simulink model "gnc_uav_toolbox_DCIntegration"  (R2025b)
settings: Solver=FixedStepAuto  StartTime=0  StopTime=cfg.stopTime  MaxStep=0.01  RelTol=1e-5
values from neighbouring files (symbols this model uses):
  C = [cfg.kPos;cfg.vNom;cfg.vMax;cfg.landSpeed;cfg.aMax ... (first row only)    [gn_init.m]    (also in gnc_init_dcintegration.m = [cfg.kPos;cfg.vNom;cfg.vMax;cfg.landSpeed;cfg.aMax;       cf; smooth_path.m = q(:, c) - Lt(c)*x + r*y)
  entryPoint = S(1,:).'    [gn_buildSearch.m]    (also in gn_build_mission.m = mission.p_end(:, 2))
  homeAir = [cfg.home(1); cfg.home(2); -cfg.altitude]    [gn_buildSearch.m]    (also in gn_build_mission.m = mission.p_end(:, 1))
  lastPoint = S(end,:).'    [gn_buildSearch.m]    (also in gn_build_mission.m = mission.p_end(:, 3))
  searchW = [wp(:, 2:n); -cfg.altitude*ones(1, n-1)]'    [gn_build_mission.m]
undefined symbols (not defined in the file or in its folder): cfg, DiscIntNeverNeededParam
libraries: uavalgslib x1, uavutilslib x1
settings Model: Creator=andrei  LastModifiedBy=andrei
settings OptimizationCC: OptimizeBlockIOStorage=off  ZeroExternalMemoryAtStartup=off  ZeroInternalMemoryAtStartup=off  OptimizeDataStoreBuffers=off  BusAssignmentInplaceUpdate=off
settings DebuggingCC: SFUnexpectedBacktrackingDiag=warning  SFNoUnconditionalDefaultTransitionDiag=warning
settings RTWCC: GenerateReport=on  BuildConfiguration=Debug  LaunchReport=on  TargetLang=C++
settings CodeAppCC: ForceParamTrailComments=on  MATLABSourceComments=on  EnableCustomComments=on
settings GRTTargetCC: MultiInstanceErrorCode=Warning  TargetLangStandard=C++11 (ISO)  CombineSignalStateStructs=on  CodeInterfacePackaging=C++ class  SubcomponentCodeInterfacePackaging=C++ class  SupportVariableSizeSignals=on

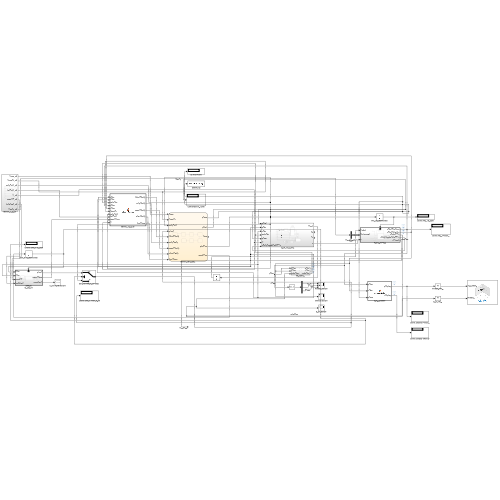
[thumbnail: Simulink's stored preview of the top-level diagram]
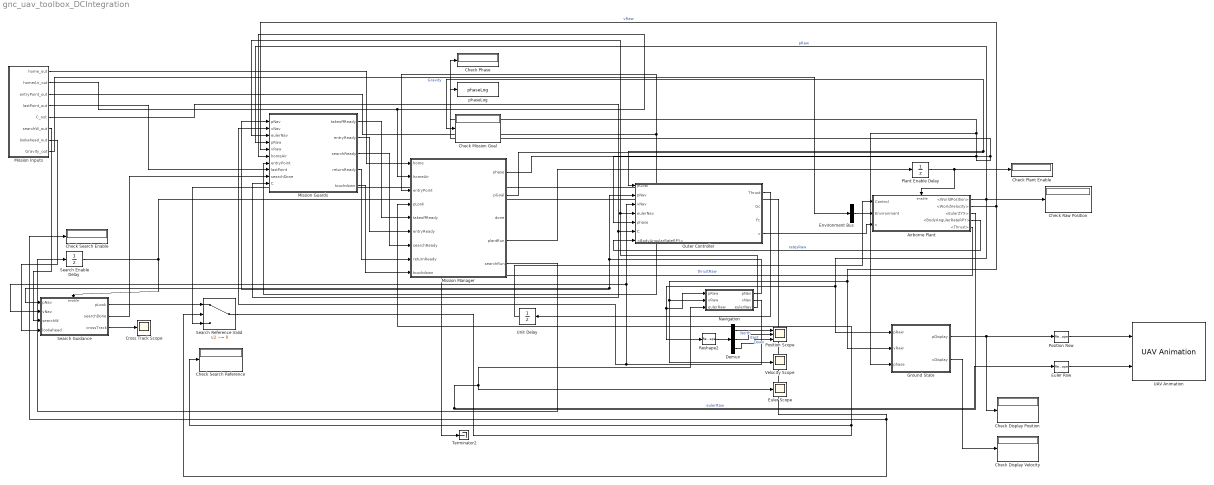
== system gnc_uav_toolbox_DCIntegration ==
  Airborne Plant : Subsystem
      settings: MinAlgLoopOccurrences=on
  Check Display Position : Display
  Check Display Velocity : Display
  Check Mission Goal : Display
  Check Phase : Display
  Check Plant Enable : Display
  Check Raw Position : Display
  Check Search Enable : Display
  Check Search Reference : Display
  Cross Track Scope : Scope
      settings: DataLoggingVariableName=ScopeData3
  Demux : Demux  Outputs=3
  Environment Bus : BusCreator  Inputs=1  OutDataTypeStr=Bus: GNEnvironmentBus  NonVirtualBus=on
  Euler Row : Reshape  OutputDimensionality=Customize  OutputDimensions=[1 3]
  Euler Scope : Scope
      settings: DataLoggingVariableName=ScopeData2
  Ground State : MATLAB Function  TreatAsAtomicUnit=on
  Mission Guards : MATLAB Function  TreatAsAtomicUnit=on
  Mission Inputs : Subsystem
  Mission Manager : Stateflow chart  TreatAsAtomicUnit=on
  Navigation : Subsystem
  Outer Controller : Subsystem
  Plant Enable Delay : UnitDelay  InitialCondition=false  SampleTime=cfg.ctrlTs  HasFrameUpgradeWarning=on
  Position Row : Reshape  OutputDimensionality=Customize  OutputDimensions=[1 3]
  Position Scope : Scope  NumInputPorts=3
      settings: ActiveDisplayYMinimum=-36.831864712326947  ActiveDisplayYMaximum=14.10248446170346
  Reshape2 : Reshape
  Search Guidance : Subsystem  TreatAsAtomicUnit=on
  Search Enable Delay : UnitDelay  InitialCondition=false  SampleTime=cfg.ctrlTs  HasFrameUpgradeWarning=on
  Search Reference Valid : Switch  Criteria=u2 ~= 0  SaturateOnIntegerOverflow=off  InputSameDT=off
  Terminator2 : Terminator
  UAV Animation : uavutilslib/UAV Animation  NumUAV=1  DynamicUAVConfig=off  UAVType=Multirotor  UAVSize=0.3  UAVColor=[0 0.45 0.74]  UAVTrajectoryAlpha=1  InertialZDirection=Down  RotationFormat=Euler ZYX  DrawMarkers=off  SampleTime=cfg.animTs
  Unit Delay : UnitDelay  InitialCondition=(cfg.mass*cfg.g/4)*ones(4,1)  SampleTime=cfg.ctrlTs  HasFrameUpgradeWarning=on
  Velocity Scope : Scope
      settings: ActiveDisplayYMinimum=-2.4801881496796212  ActiveDisplayYMaximum=2.1396138851515727
  phaseLog : ToWorkspace  VariableName=phaseLog  SaveFormat=Timeseries  SampleTime=cfg.ctrlTs
  wires:
  Navigation/1(pNav) -> Mission Guards/1(pNav), Search Guidance/1(pNav), Outer Controller/2(pNav)
  Navigation/2(vNav) -> Mission Guards/2(vNav), Outer Controller/3(vNav), Search Guidance/2(vNav)
  Navigation/3(eulerNav) -> Mission Guards/3(eulerNav), Outer Controller/4(eulerNav)
  Reshape2/1 -> Demux/1
  Demux/1 -> Position Scope/1  "North"
  Demux/2 -> Position Scope/2  "East"
  Demux/3 -> Position Scope/3  "Down"
  Search Enable Delay/1 -> Search Reference Valid/2, Check Search Enable/1, Search Guidance/Enable
  Search Guidance/1(pLook) -> Search Reference Valid/1
  Search Guidance/2(searchDone) -> Mission Guards/9(searchDone)
  Mission Guards/1(takeoffReady) -> Mission Manager/5(takeoffReady)
  Mission Guards/2(entryReady) -> Mission Manager/6(entryReady)
  Mission Guards/3(searchReady) -> Mission Manager/7(searchReady)
  Mission Guards/4(returnReady) -> Mission Manager/8(returnReady)
  Mission Guards/5(touchdown) -> Mission Manager/9(touchdown)
  Airborne Plant/2(<WorldVelocity>) -> Navigation/2(vRaw), Velocity Scope/1, Ground State/2(vRaw), Mission Guards/5(vRaw)  "vRaw"
  Airborne Plant/3(<EulerZYX>) -> Euler Scope/1, Navigation/3(eulerRaw), Euler Row/1  "eulerRaw"
  Airborne Plant/1(<WorldPosition>) -> Check Raw Position/1, Mission Guards/4(pRaw), Ground State/1(pRaw), Navigation/1(pRaw), Reshape2/1  "pRaw"
  Environment Bus/1 -> Airborne Plant/2(Environment)
  Airborne Plant/4(<BodyAngularRateRPY>) -> Outer Controller/7(<BodyAngularRateRPY>)  "ratesRaw"
  Airborne Plant/5(<Thrust>) -> Terminator2/1  "thrustRaw"
  Plant Enable Delay/1 -> Airborne Plant/Enable, Check Plant Enable/1
  Mission Manager/4(plantRun) -> Plant Enable Delay/1
  Mission Manager/5(searchRun) -> Search Enable Delay/1
  Search Reference Valid/1 -> Check Search Reference/1, Mission Manager/4(pLook)
  Mission Manager/1(phase) -> phaseLog/1, Outer Controller/5(phase), Check Phase/1, Ground State/3(phase)
  Ground State/2(vDisplay) -> Check Display Velocity/1
  Ground State/1(pDisplay) -> Check Display Position/1, Position Row/1
  Mission Manager/2(pGoal) -> Outer Controller/1(pGoal), Check Mission Goal/1
  Mission Inputs/2(homeAir_out) -> Mission Guards/6(homeAir), Mission Manager/2(homeAir)
  Mission Inputs/3(entryPoint_out) -> Mission Guards/7(entryPoint), Search Reference Valid/3, Mission Manager/3(entryPoint)
  Mission Inputs/5(C_out) -> Mission Guards/10(C), Outer Controller/6(C)
  Mission Inputs/1(home_out) -> Mission Manager/1(home)
  Mission Inputs/4(lastPoint_out) -> Mission Guards/8(lastPoint)
  Mission Inputs/6(searchW_out) -> Search Guidance/3(searchW)
  Mission Inputs/7(lookahead_out) -> Search Guidance/4(lookahead)
  Mission Inputs/8(Gravity_out) -> Environment Bus/1  "Gravity"
  Search Guidance/3(crossTrack) -> Cross Track Scope/1
  Position Row/1 -> UAV Animation/1
  Euler Row/1 -> UAV Animation/2
  Outer Controller/1(Thrust) -> Unit Delay/1
  Outer Controller/4(c) -> Airborne Plant/3(c)
  Unit Delay/1 -> Airborne Plant/1(Control)

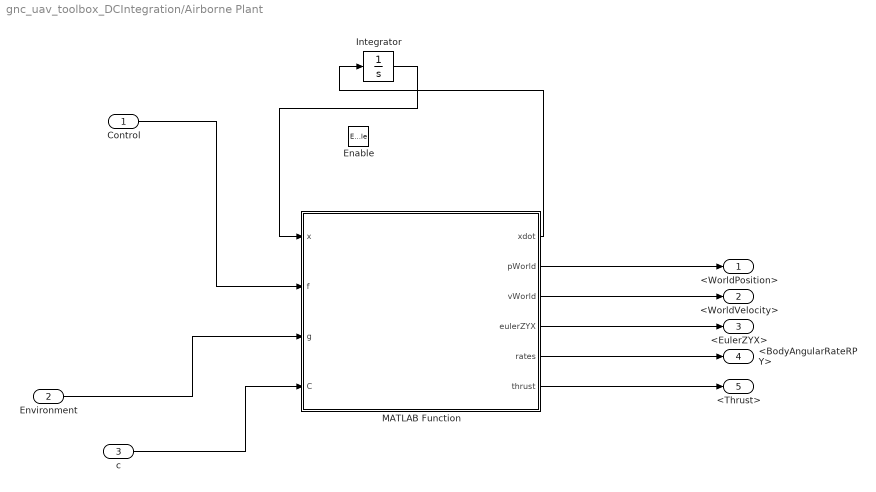
== system gnc_uav_toolbox_DCIntegration/Airborne Plant ==
  Control : Inport
  Environment : Inport  Port=2
  c : Inport  Port=3
  Enable : EnablePort
  Integrator : Integrator
  MATLAB Function : MATLAB Function  TreatAsAtomicUnit=on
  <WorldPosition> : Outport
  <WorldVelocity> : Outport  Port=2
  <EulerZYX> : Outport  Port=3
  <BodyAngularRateRPY> : Outport  Port=4
  <Thrust> : Outport  Port=5
  wires:
  MATLAB Function/5(rates) -> <BodyAngularRateRPY>/1
  Environment/1 -> MATLAB Function/3(g)
  MATLAB Function/6(thrust) -> <Thrust>/1
  MATLAB Function/2(pWorld) -> <WorldPosition>/1
  Control/1 -> MATLAB Function/2(f)
  MATLAB Function/4(eulerZYX) -> <EulerZYX>/1
  MATLAB Function/3(vWorld) -> <WorldVelocity>/1
  MATLAB Function/1(xdot) -> Integrator/1
  Integrator/1 -> MATLAB Function/1(x)
  c/1 -> MATLAB Function/4(C)

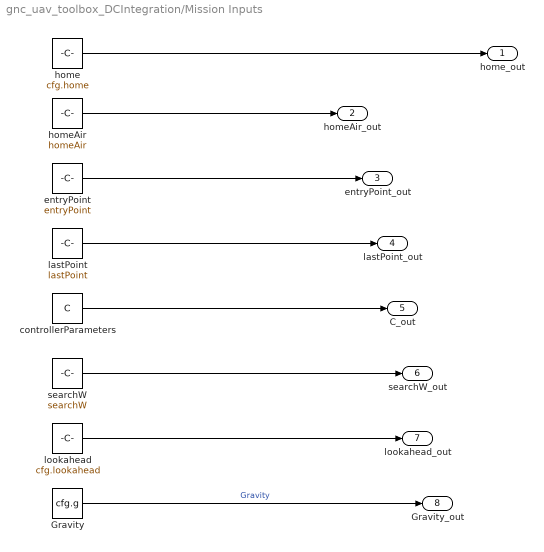
== system gnc_uav_toolbox_DCIntegration/Mission Inputs ==
  Gravity : Constant  Value=cfg.g  VectorParams1D=off
  controllerParameters : Constant  Value=C  VectorParams1D=off
  entryPoint : Constant  Value=entryPoint  VectorParams1D=off
  home : Constant  Value=cfg.home  VectorParams1D=off
  homeAir : Constant  Value=homeAir  VectorParams1D=off
  lastPoint : Constant  Value=lastPoint  VectorParams1D=off
  lookahead : Constant  Value=cfg.lookahead  VectorParams1D=off
  searchW : Constant  Value=searchW  VectorParams1D=off
  home_out : Outport
  homeAir_out : Outport  Port=2
  entryPoint_out : Outport  Port=3
  lastPoint_out : Outport  Port=4
  C_out : Outport  Port=5
  searchW_out : Outport  Port=6
  lookahead_out : Outport  Port=7
  Gravity_out : Outport  Port=8
  wires:
  searchW/1 -> searchW_out/1
  lastPoint/1 -> lastPoint_out/1
  entryPoint/1 -> entryPoint_out/1
  lookahead/1 -> lookahead_out/1
  controllerParameters/1 -> C_out/1
  homeAir/1 -> homeAir_out/1
  Gravity/1 -> Gravity_out/1  "Gravity"
  home/1 -> home_out/1

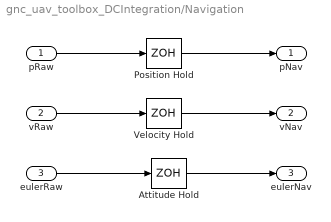
== system gnc_uav_toolbox_DCIntegration/Navigation ==
  pRaw : Inport
  vRaw : Inport  Port=2
  eulerRaw : Inport  Port=3
  Attitude Hold : ZeroOrderHold  SampleTime=cfg.ctrlTs
  Position Hold : ZeroOrderHold  SampleTime=cfg.navTs
  Velocity Hold : ZeroOrderHold  SampleTime=cfg.navTs
  pNav : Outport
  vNav : Outport  Port=2
  eulerNav : Outport  Port=3
  wires:
  pRaw/1 -> Position Hold/1
  vRaw/1 -> Velocity Hold/1
  eulerRaw/1 -> Attitude Hold/1
  Position Hold/1 -> pNav/1
  Velocity Hold/1 -> vNav/1
  Attitude Hold/1 -> eulerNav/1

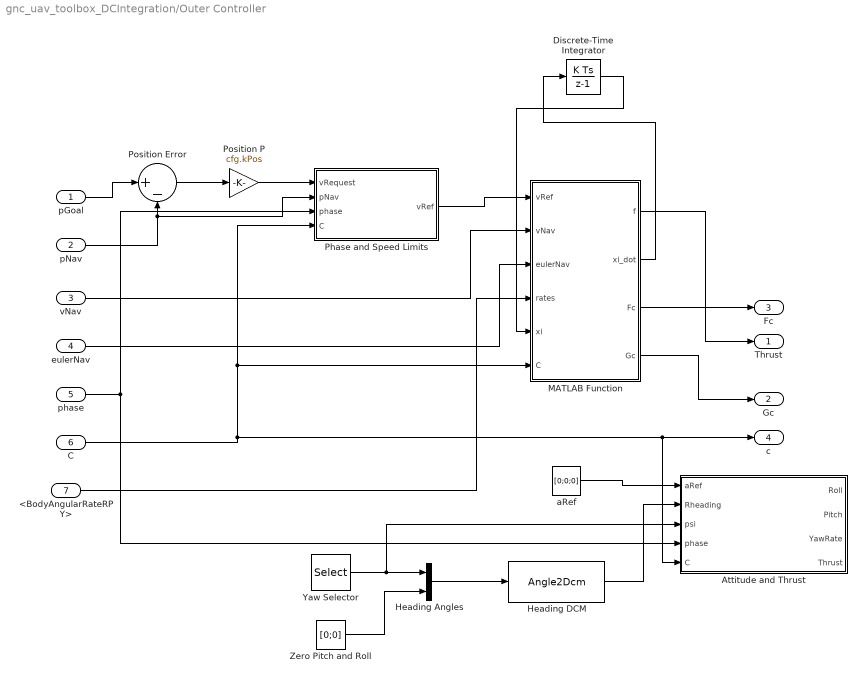
== system gnc_uav_toolbox_DCIntegration/Outer Controller ==
  pGoal : Inport
  pNav : Inport  Port=2
  vNav : Inport  Port=3
  eulerNav : Inport  Port=4
  phase : Inport  Port=5
  C : Inport  Port=6
  <BodyAngularRateRPY> : Inport  Port=7
  Attitude and Thrust : MATLAB Function  TreatAsAtomicUnit=on
  Discrete-Time Integrator : DiscreteIntegrator  SampleTime=-1  ICPrevOutput=DiscIntNeverNeededParam  ICPrevScaledInput=DiscIntNeverNeededParam
  Heading Angles : Concatenate  Mode=Multidimensional array
  Heading DCM : Angle2Dcm
      settings: AttributesFormatString=Rotation Order: %<rotationOrder>
  MATLAB Function : MATLAB Function  TreatAsAtomicUnit=on
  Phase and Speed Limits : MATLAB Function  TreatAsAtomicUnit=on
  Position Error : Sum  Inputs=|+-
  Position P : Gain  Gain=cfg.kPos
  Yaw Selector : Selector  InputPortWidth=3  IndexOptions=Index vector (dialog)  Indices=[1]  OutputSizes=1
  Zero Pitch and Roll : Constant  Value=[0;0]  VectorParams1D=off
  aRef : Constant  Value=[0;0;0]  VectorParams1D=off
  Thrust : Outport
  Gc : Outport  Port=2
  Fc : Outport  Port=3
  c : Outport  Port=4
  wires:
  pGoal/1 -> Position Error/1
  pNav/1 -> Phase and Speed Limits/2(pNav), Position Error/2
  Phase and Speed Limits/1(vRef) -> MATLAB Function/1(vRef)
  vNav/1 -> MATLAB Function/2(vNav)
  Position Error/1 -> Position P/1
  Position P/1 -> Phase and Speed Limits/1(vRequest)
  phase/1 -> Attitude and Thrust/4(phase), Phase and Speed Limits/3(phase)
  C/1 -> Phase and Speed Limits/4(C), MATLAB Function/6(C), Attitude and Thrust/5(C), c/1
  eulerNav/1 -> MATLAB Function/3(eulerNav)
  Yaw Selector/1 -> Attitude and Thrust/3(psi), Heading Angles/1
  Zero Pitch and Roll/1 -> Heading Angles/2
  Heading Angles/1 -> Heading DCM/1
  Heading DCM/1 -> Attitude and Thrust/2(Rheading)
  MATLAB Function/2(xi_dot) -> Discrete-Time Integrator/1
  Discrete-Time Integrator/1 -> MATLAB Function/5(xi)
  <BodyAngularRateRPY>/1 -> MATLAB Function/4(rates)
  MATLAB Function/1(f) -> Thrust/1
  MATLAB Function/3(Fc) -> Fc/1
  MATLAB Function/4(Gc) -> Gc/1
  aRef/1 -> Attitude and Thrust/1(aRef)

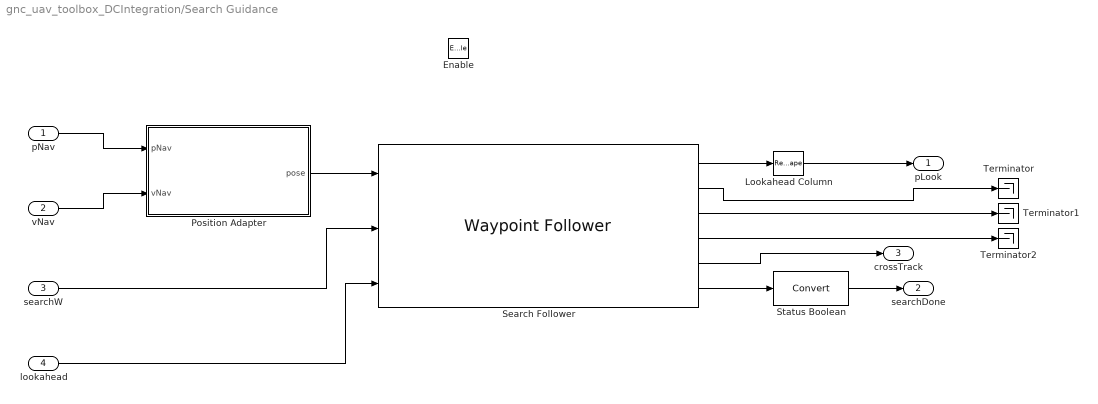
== system gnc_uav_toolbox_DCIntegration/Search Guidance ==
  pNav : Inport
  vNav : Inport  Port=2
  searchW : Inport  Port=3
  lookahead : Inport  Port=4
  Enable : EnablePort
  Lookahead Column : Reshape  OutputDimensionality=Column vector (2-D)
  Position Adapter : MATLAB Function  TreatAsAtomicUnit=on
  Search Follower : uavalgslib/Waypoint Follower  UAVType=multirotor  StartFrom=first  TransitionRadiusSource=internal  TransitionRadius=cfg.transitionRadius  MinLookaheadDistance=0.1  HoverAtLastWaypoint=on  YawInput=off  ShowCrossTrackErrorOutput=on  ShowStatusOutput=on  SimulateUsing=Interpreted execution
  Status Boolean : DataTypeConversion  SaturateOnIntegerOverflow=off  RndMeth=Floor
  Terminator : Terminator
  Terminator1 : Terminator
  Terminator2 : Terminator
  pLook : Outport  OutputWhenDisabled=reset  InitialOutput=[0;0;0]
  searchDone : Outport  Port=2  OutputWhenDisabled=reset  InitialOutput=[false]
  crossTrack : Outport  Port=3  OutputWhenDisabled=reset  InitialOutput=[0]
  wires:
  pNav/1 -> Position Adapter/1(pNav)
  vNav/1 -> Position Adapter/2(vNav)
  Position Adapter/1(pose) -> Search Follower/1
  searchW/1 -> Search Follower/2
  lookahead/1 -> Search Follower/3
  Search Follower/1 -> Lookahead Column/1
  Lookahead Column/1 -> pLook/1
  Search Follower/6 -> Status Boolean/1
  Status Boolean/1 -> searchDone/1
  Search Follower/5 -> crossTrack/1
  Search Follower/4 -> Terminator2/1
  Search Follower/3 -> Terminator1/1
  Search Follower/2 -> Terminator/1

== matlab function gnc_uav_toolbox_DCIntegration/Ground State ==
  settings: updateMethod=DISCRETE  sampleTime=cfg.ctrlTs
  data: pRaw input; pDisplay output; vRaw input; phase input; vDisplay output
function [pDisplay,vDisplay] = groundState(pRaw,vRaw,phase)
% Position and velocity for display and landed reporting.

% Normally report the unmodified plant state.
pDisplay = pRaw;
vDisplay = vRaw;

% During PRECHECK or COMPLETE, report the vehicle on the ground.
if phase == 0 || phase == 6
    pDisplay(3) = 0;
    vDisplay = zeros(3,1);
end
end

== matlab function gnc_uav_toolbox_DCIntegration/Outer Controller/MATLAB Function ==
  data: vRef input; f output double size=[4 1]; vNav input; eulerNav input; rates input; xi input; C input; xi_dot output double size=[5 1]; Fc output double size=[3 1]; Gc output double size=[3 1]
function [f, xi_dot, Fc, Gc] = DCController(vRef, vNav, eulerNav, rates, xi, C)
% DCController - D&C inner part of 'Outer Controller'. Replaces Velocity P,
% limitAcceleration and accelToCommands. Keep Position P + limitVelocity
% (mission-phase logic) upstream; vRef is limitVelocity's output (NED, m/s).
% eulerNav = [psi; theta; phi] (ZYX order). xi = [xi_phi xi_theta xi_u xi_v xi_z]'.
% C = parameter vector from gn_init:
%   C(5) aMax, C(6) m, C(7) g, C(8) tiltMax, C(12:14) Ix Iy Iz, C(15) d,
%   C(16) km, C(19) f_max, C(20:25) kpu kiu kpv kiv kpw kiw
aMax=C(5); m=C(6); g=C(7); tilt=C(8);
Ix=C(12); Iy=C(13); Iz=C(14); d=C(15); km=C(16); f_max=C(19);
kpu=C(20); kiu=C(21); kpv=C(22); kiv=C(23); kpw=C(24); kiw=C(25);
 
psi=eulerNav(1); theta=eulerNav(2); phi=eulerNav(3);
p=rates(1); q=rates(2); r=rates(3);
cph=cos(phi); cth=cos(theta); cps=cos(psi); sps=sin(psi);
psiRef = 0;
 
ex = vNav(1)-vRef(1); ey = vNav(2)-vRef(2); ez = vNav(3)-vRef(3);
xdd = -kpu*ex - kiu*xi(3);
ydd = -kpv*ey - kiv*xi(4);
zdd = -kpw*ez - kiw*xi(5);
 
% Acceleration-norm limit (same rule as the lead's limitAcceleration)
s = sqrt(xdd^2 + ydd^2 + zdd^2);
a_sat = s > aMax;
if a_sat
    k = aMax/s;
    xdd = xdd*k; ydd = ydd*k; zdd = zdd*k;
end
 
axH =  cps*xdd + sps*ydd;
ayH = -sps*xdd + cps*ydd;
th_raw = -axH/g;  ph_raw = ayH/g;
th_ref = max(min(th_raw, tilt), -tilt);
ph_ref = max(min(ph_raw, tilt), -tilt);
tcos  = max(cph*cth, cos(tilt + deg2rad(15)));
T_cmd = m*(g - zdd)/tcos;
T_max = 4*f_max;
T = max(min(T_cmd, T_max), 0);
Fc = [0; 0; -T];
 
x_sat = abs(th_raw) >= tilt || a_sat;
y_sat = abs(ph_raw) >= tilt || a_sat;
z_sat = (T_cmd > T_max && ez > 0) || (T_cmd < 0 && ez < 0) || a_sat;
 
l1=-1/0.5; l2=-1/0.05; l3=-1/1;
e2 = l1*l2 + l1*l3 + l2*l3;  e1 = -(l1+l2+l3);  e0 = -l1*l2*l3;
phi_err = phi - ph_ref;  theta_err = theta - th_ref;
psi_err = atan2(sin(psi-psiRef), cos(psi-psiRef));
kp_yaw = Iz*(1/0.5)*(1/0.2);  kd_yaw = Iz*(1/0.5 + 1/0.2);
L = -Ix*e2*phi_err   - Ix*e1*p - Ix*e0*xi(1);
M = -Iy*e2*theta_err - Iy*e1*q - Iy*e0*xi(2);
N = -kp_yaw*psi_err  - kd_yaw*r;
Gc = [L; M; N];
xi_dot = [phi_err; theta_err; ex*~x_sat; ey*~y_sat; ez*~z_sat];
 
T  = -Fc(3);
Lp = Gc(1)/(d/sqrt(2));
Mp = Gc(2)/(d/sqrt(2));
Np = Gc(3)/km;

% Explicitly allocate four motor thrust outputs
f = zeros(4,1);

f(1) = 0.25*(T - Lp + Mp + Np);
f(2) = 0.25*(T - Lp - Mp - Np);
f(3) = 0.25*(T + Lp - Mp + Np);
f(4) = 0.25*(T + Lp + Mp - Np);

% Saturate individual motor thrusts
for i = 1:4
    f(i) = max(0, min(f(i), f_max));
end
end

== matlab function gnc_uav_toolbox_DCIntegration/Airborne Plant/MATLAB Function ==
  data: x input size=[12 1]; xdot output size=[12 1]; f input size=[4 1]; g input size=[1 1]; C input size=[25 1]; pWorld output size=[3 1]; vWorld output size=[3 1]; eulerZYX output size=[3 1]; rates output size=[3 1]; thrust output size=[1 1]
function [xdot, pWorld, vWorld, eulerZYX, rates, thrust] = DCPlantMotors(x, f, g, C)
% DCPlantMotors - 6-DOF quadrotor body driven by the four motor forces f.
% Use with DCController's f output (carries the per-motor [0,f_max] clamp).
% x = [xE yE zE phi theta psi uB vB wB p q r]. Feed xdot to an Integrator
% (IC = [home(:); zeros(9,1)]) and its output back into x.
% C = parameter vector from gn_init (set C as a block Parameter):
%   C(6) m, C(7) g, C(12:14) Ix Iy Iz, C(15) d, C(16) km, C(17) nu, C(18) mu
m=C(6); g=C(7); Ix=C(12); Iy=C(13); Iz=C(14);
d=C(15); km=C(16); nu=C(17); mu=C(18);
 
phi=x(4); theta=x(5); psi=x(6);
uB=x(7); vB=x(8); wB=x(9); p=x(10); q=x(11); r=x(12);
Zc = -(f(1)+f(2)+f(3)+f(4));
a  = d/sqrt(2);
Lc = a*(-f(1)-f(2)+f(3)+f(4));
Mc = a*( f(1)-f(2)-f(3)+f(4));
Nc = km*(f(1)-f(2)+f(3)-f(4));
X = -nu*uB*abs(uB);  Y = -nu*vB*abs(vB);  Z = Zc - nu*wB*abs(wB);
L = Lc - mu*p*abs(p); M = Mc - mu*q*abs(q); N = Nc - mu*r*abs(r);
cph=cos(phi); sph=sin(phi); cth=cos(theta); sth=sin(theta); cps=cos(psi); sps=sin(psi);
tth = tan(theta); sec_th = 1/cth;
xdot = [ cth*cps*uB + (sph*sth*cps - cph*sps)*vB + (cph*sth*cps + sph*sps)*wB;
         cth*sps*uB + (sph*sth*sps + cph*cps)*vB + (cph*sth*sps - sph*cps)*wB;
        -sth*uB + sph*cth*vB + cph*cth*wB;
         p + sph*tth*q + cph*tth*r;
         cph*q - sph*r;
         sph*sec_th*q + cph*sec_th*r;
         r*vB - q*wB - g*sth     + X/m;
         p*wB - r*uB + g*cth*sph + Y/m;
         q*uB - p*vB + g*cth*cph + Z/m;
         (L + (Iy-Iz)*q*r)/Ix;
         (M + (Iz-Ix)*p*r)/Iy;
         (N + (Ix-Iy)*p*q)/Iz ];
pWorld=x(1:3); vWorld=xdot(1:3); eulerZYX=[psi;theta;phi]; rates=[p;q;r]; thrust=-Zc;
end

== matlab function gnc_uav_toolbox_DCIntegration/Outer Controller/Phase and Speed Limits ==
  settings: updateMethod=DISCRETE  sampleTime=cfg.ctrlTs
  data: vRequest input; vRef output; pNav input; phase input; C input
function vRef = limitVelocity(vRequest,pNav,phase,C)

vRef=vRequest;

if phase==0 || phase==6

    vRef=zeros(3,1);

elseif phase==1

    vRef(1:2)=0;

elseif phase==5

    vRef=zeros(3,1);

    vRef(3)=min(C(4),max(0.03,C(1)*max(0,-pNav(3))));

end

s=norm(vRef); limit=min(C(2),C(3));

if s>limit

    vRef=vRef*(limit/s);

end

end

== matlab function gnc_uav_toolbox_DCIntegration/Outer Controller/Attitude and Thrust ==
  settings: updateMethod=DISCRETE  sampleTime=cfg.ctrlTs
  data: Roll output; Pitch output; YawRate output; Thrust output; aRef input size=[3 1]; Rheading input size=[3 3]; psi input size=[1 1]; phase input size=[1 1]; C input size=[25 1]
function [Roll,Pitch,YawRate,Thrust] = accelToCommands(aRef,Rheading,psi,phase,C)

m=C(6); g=C(7); tiltMax=C(8);

aHeading=Rheading*aRef;

verticalSupport=max(0.5*g,g-aHeading(3));

supportNorm=sqrt(aHeading(1)^2+aHeading(2)^2+verticalSupport^2);

Roll=asin(max(-1,min(1,aHeading(2)/supportNorm)));

Pitch=atan2(-aHeading(1),verticalSupport);

Roll=max(-tiltMax,min(tiltMax,Roll));

Pitch=max(-tiltMax,min(tiltMax,Pitch));

Thrust=m*verticalSupport/max(0.2,cos(Roll)*cos(Pitch));

Thrust=max(0,min(2*m*g,Thrust));

YawRate=max(-0.3,min(0.3,-psi));

if phase==0 || phase==6

    Roll=0; Pitch=0; YawRate=0; Thrust=0;

end

end

== matlab function gnc_uav_toolbox_DCIntegration/Search Guidance/Position Adapter ==
  data: pNav input double size=[3 1]; pose output double size=[4 1]; vNav input double size=[3 1]
function pose = makeFollowerPose(pNav,vNav)

if hypot(vNav(1),vNav(2))>1e-4

    chi=atan2(vNav(2),vNav(1));

else

    chi=0;

end

pose=[pNav;chi];

end

== matlab function gnc_uav_toolbox_DCIntegration/Mission Guards ==
  settings: updateMethod=DISCRETE  sampleTime=cfg.ctrlTs
  data: pNav input; takeoffReady output; vNav input; eulerNav input; pRaw input; vRaw input; homeAir input; entryPoint input; lastPoint input; searchDone input; C input; entryReady output; searchReady output; returnReady output; touchdown output
function [takeoffReady,entryReady,searchReady,returnReady, touchdown] = missionGuards(pNav,vNav,eulerNav,pRaw,vRaw,homeAir, entryPoint,lastPoint,searchDone,C)
slow=norm(vNav)<=C(11);
takeoffReady=norm(pNav-homeAir)<=C(9) && slow;
entryReady=norm(pNav-entryPoint)<=C(9) && slow;
searchReady=searchDone && norm(pNav-lastPoint)<=C(9) && slow;
level=abs(eulerNav(2))<=deg2rad(1) && abs(eulerNav(3))<=deg2rad(1);
returnReady=norm(pNav-homeAir)<=C(10) && slow && level;
touchdown=pRaw(3)>=0 && vRaw(3)>=-0.02;
end

== stateflow chart gnc_uav_toolbox_DCIntegration/Mission Manager ==
  settings: updateMethod=DISCRETE  sampleTime=cfg.ctrlTs
  state PRECHECK
    entry, during:
    phase=0;
    pGoal=home;
    done=false;
    plantRun=false;
    searchRun=false;
  state TRANSIT
    entry, during:
    phase=2;
    pGoal=entryPoint;
    done=false;
    plantRun=true;
    searchRun=false;
  state SEARCH
    entry, during:
    phase=3;
    pGoal=pLook;
    done=false;
    plantRun=true;
    searchRun=true;
  state TAKEOFF
    entry, during:
    phase=1;
    pGoal=homeAir;
    done=false;
    plantRun=true;
    searchRun=false;
  state RETURN
    entry, during:
    phase=4;
    pGoal=homeAir;
    done=false;
    plantRun=true;
    searchRun=false;
  state COMPLETE
    entry, during:
    phase=6;
    pGoal=home;
    done=true;
    plantRun=false;
    searchRun=false;
  state LAND
    entry, during:
    phase=5;
    pGoal=home;
    done=false;
    plantRun=true;
    searchRun=false;
  (default) -> PRECHECK
  PRECHECK -> TAKEOFF : after(1,sec)
  TAKEOFF -> TRANSIT : [takeoffReady]
  TRANSIT -> SEARCH : [entryReady]
  SEARCH -> RETURN : [searchReady]
  RETURN -> LAND : [returnReady]
  LAND -> COMPLETE : [touchdown]
  data: home input double size=[3, 1]; homeAir input double size=[3, 1]; entryPoint input double size=[3, 1]; pLook input double size=[3, 1]; takeoffReady input boolean size=1; entryReady input boolean size=1; searchReady input boolean size=1; returnReady input boolean size=1; touchdown input boolean size=1; phase output double size=1; pGoal output double size=[3, 1]; done output boolean size=1; plantRun output boolean size=1; searchRun output boolean size=1
